simulink model "furuta_block_model_fixed_ppo_swingup"  (R2026b)
settings: Solver=ode14x  StopTime=25  FixedStep=driveElectrical.sampleTime
InitFcn:
  | validate_furuta_fixed_test(bdroot);
model workspace (MAT data in the model file):
  calibration = [73.65 -1 4058.5 1]
  controlPeriod = 0.01
  drive = [-1 1.5 1.5 inf]
  driveElectrical : object (value not decoded)
  failureReplayEnabled = 0
  failureReplaySlowdown = 10
  failureReplaySource = 'C:\Capstone1\matlab_furuta\results\ppo_rmd_candidate_tpa79dc374_f9fe_4d66_a12a_2e210f4a8415\ppo_start_-20_+20_armrate_20_current_1.5_time_10_armlimit_Inf.mat'
  failureReplayStartDeg = 20
  failureReplayState = [0 0.1 0.2 0.3 0.4 0.5 0.6 0.7 0.8 0.9 1 1.1 ... (205 elements, 41x5)]
  furutaPPOAgent : rl.agent.rlPPOAgent (value not decoded)
  furutaSACAgent : rl.agent.rlSACAgent (value not decoded)
  furutaToolboxMpc : object (value not decoded)
  initialState = [0; 3.14159265359; 0; 0]
  integrationStep = 0.002
  limits = [inf 3.3 15 20]
  lqrGain = [-1.90684760658 -25.0276005412 -1.03983138576 -2.50199272238]
  maxTorque = 3.15
  milVelocityLimits = [15 25]
  pidGains = [25.0276005412 5.00398544475 1.90684760658 2.07966277151 0.001]
  plantCoefficients = [0.05 0.00016078 0.00016134 0.00013805 0.016934 0.0001 1e-05 0.63]
  rlRewardLevel = 2
  rmd : object (value not decoded)
  rmdCommandDelaySamples = 1
  scenarioStimulus = [0  0  0  0; 20  0  0  0]
  swingLqrThresholds = [0.226892802759 0.2 0.523598775598]
  usePolicyCallback = 0
  useRmd = 1
  velocityFilterTau = 0.03
values from neighbouring files (symbols this model uses):
  C = [B A*B A^2*B A^3*B]    [build_furuta_rmd.m]
  N = 20    [build_furuta_rl.m]    (also in design_classical.m)
  s = load(matFile,'ds')    [analyze_pi_current_run.m]    (also in analyze_pi_speed_run.m; build_furuta_rl.m = sin(x(2));"; build_furuta_simulink.m = s(1); design_classical.m = furuta_scenarios)
  source = [step '/1']    [add_furuta_plant_blocks.m]    (also in build_furuta_pi.m = get_param(line,'SrcPortHandle'); build_furuta_pi_hardware.m = 'Drive interlocks/3'; compare_furuta_actuators.m = get_param([harness '/Requested torque'],'PortHandles'))
  Z = expm([A B; zeros(1,5)]*p.Ts)    [furuta_linearize.m]
symbols that are objects in the model workspace (value not decoded): driveElectrical, rmd
undefined symbols (not defined in the file or in its folder): lmpcF, lmpcH, poleGain, sgn, X, Y
libraries: sm_lib x36, raspberrypiCommlib x9, nesl_utility x8, fl_lib x7, rllib x2, mpclib x1, slpidlib x1, ee_lib x1
(part 4 of 4)

== system furuta_block_model_fixed_ppo_swingup/01 MIL - Controller and Plant/05 Furuta plant/RK4 Furuta plant/Substep 4/k3 ==
  x : Inport
  tau : Inport  Port=2
  Arm acceleration : Fcn  Expr=(u(3)*u(4)-u(2)*u(5))/(u(1)*u(3)-(u(2)*u(2)))
  Arm rate : Fcn  Expr=u(3)
  D11 : Fcn  Expr=u(6)+u(7)*(sin(u(2))*sin(u(2)))
  D12 : Fcn  Expr=u(9)*cos(u(2))
  D22 : Fcn  Expr=u(8)
  Mass matrix and RHS : Mux  Inputs=5
  Pend acceleration : Fcn  Expr=(u(1)*u(5)-u(2)*u(4))/(u(1)*u(3)-(u(2)*u(2)))
  Pend rate : Fcn  Expr=u(4)
  Physical parameters : Constant  Value=plantCoefficients
  State derivative : Mux
  State torque parameters : Mux  Inputs=3
  Torque RHS arm : Fcn  Expr=u(5)-2*u(7)*sin(u(2))*cos(u(2))*u(3)*u(4)+u(9)*sin(u(2))*(u(4)*u(4))-u(11)*u(3)-u(13)*sgn(u(3))
  Torque RHS pend : Fcn  Expr=u(7)*sin(u(2))*cos(u(2))*(u(3)*u(3))-u(12)*u(4)+u(10)*sin(u(2))
  xdot : Outport
  wires:
  x/1 -> State torque parameters/1
  tau/1 -> State torque parameters/2
  Physical parameters/1 -> State torque parameters/3
  State torque parameters/1 -> Arm rate/1, Pend rate/1, Torque RHS pend/1, Torque RHS arm/1, D22/1, D11/1, D12/1
  D11/1 -> Mass matrix and RHS/1
  D12/1 -> Mass matrix and RHS/2
  D22/1 -> Mass matrix and RHS/3
  Torque RHS arm/1 -> Mass matrix and RHS/4
  Torque RHS pend/1 -> Mass matrix and RHS/5
  Arm rate/1 -> State derivative/1
  Pend rate/1 -> State derivative/2
  Mass matrix and RHS/1 -> Arm acceleration/1, Pend acceleration/1
  Arm acceleration/1 -> State derivative/3
  Pend acceleration/1 -> State derivative/4
  State derivative/1 -> xdot/1

== system furuta_block_model_fixed_ppo_swingup/01 MIL - Controller and Plant/05 Furuta plant/RK4 Furuta plant/Substep 4/k4 ==
  x : Inport
  tau : Inport  Port=2
  Arm acceleration : Fcn  Expr=(u(3)*u(4)-u(2)*u(5))/(u(1)*u(3)-(u(2)*u(2)))
  Arm rate : Fcn  Expr=u(3)
  D11 : Fcn  Expr=u(6)+u(7)*(sin(u(2))*sin(u(2)))
  D12 : Fcn  Expr=u(9)*cos(u(2))
  D22 : Fcn  Expr=u(8)
  Mass matrix and RHS : Mux  Inputs=5
  Pend acceleration : Fcn  Expr=(u(1)*u(5)-u(2)*u(4))/(u(1)*u(3)-(u(2)*u(2)))
  Pend rate : Fcn  Expr=u(4)
  Physical parameters : Constant  Value=plantCoefficients
  State derivative : Mux
  State torque parameters : Mux  Inputs=3
  Torque RHS arm : Fcn  Expr=u(5)-2*u(7)*sin(u(2))*cos(u(2))*u(3)*u(4)+u(9)*sin(u(2))*(u(4)*u(4))-u(11)*u(3)-u(13)*sgn(u(3))
  Torque RHS pend : Fcn  Expr=u(7)*sin(u(2))*cos(u(2))*(u(3)*u(3))-u(12)*u(4)+u(10)*sin(u(2))
  xdot : Outport
  wires:
  x/1 -> State torque parameters/1
  tau/1 -> State torque parameters/2
  Physical parameters/1 -> State torque parameters/3
  State torque parameters/1 -> Arm rate/1, Pend rate/1, Torque RHS pend/1, Torque RHS arm/1, D22/1, D11/1, D12/1
  D11/1 -> Mass matrix and RHS/1
  D12/1 -> Mass matrix and RHS/2
  D22/1 -> Mass matrix and RHS/3
  Torque RHS arm/1 -> Mass matrix and RHS/4
  Torque RHS pend/1 -> Mass matrix and RHS/5
  Arm rate/1 -> State derivative/1
  Pend rate/1 -> State derivative/2
  Mass matrix and RHS/1 -> Arm acceleration/1, Pend acceleration/1
  Arm acceleration/1 -> State derivative/3
  Pend acceleration/1 -> State derivative/4
  State derivative/1 -> xdot/1

== system furuta_block_model_fixed_ppo_swingup/01 MIL - Controller and Plant/05 Furuta plant/RK4 Furuta plant/Substep 5/k1 ==
  x : Inport
  tau : Inport  Port=2
  Arm acceleration : Fcn  Expr=(u(3)*u(4)-u(2)*u(5))/(u(1)*u(3)-(u(2)*u(2)))
  Arm rate : Fcn  Expr=u(3)
  D11 : Fcn  Expr=u(6)+u(7)*(sin(u(2))*sin(u(2)))
  D12 : Fcn  Expr=u(9)*cos(u(2))
  D22 : Fcn  Expr=u(8)
  Mass matrix and RHS : Mux  Inputs=5
  Pend acceleration : Fcn  Expr=(u(1)*u(5)-u(2)*u(4))/(u(1)*u(3)-(u(2)*u(2)))
  Pend rate : Fcn  Expr=u(4)
  Physical parameters : Constant  Value=plantCoefficients
  State derivative : Mux
  State torque parameters : Mux  Inputs=3
  Torque RHS arm : Fcn  Expr=u(5)-2*u(7)*sin(u(2))*cos(u(2))*u(3)*u(4)+u(9)*sin(u(2))*(u(4)*u(4))-u(11)*u(3)-u(13)*sgn(u(3))
  Torque RHS pend : Fcn  Expr=u(7)*sin(u(2))*cos(u(2))*(u(3)*u(3))-u(12)*u(4)+u(10)*sin(u(2))
  xdot : Outport
  wires:
  State derivative/1 -> xdot/1
  Pend acceleration/1 -> State derivative/4
  Arm acceleration/1 -> State derivative/3
  Mass matrix and RHS/1 -> Pend acceleration/1, Arm acceleration/1
  Pend rate/1 -> State derivative/2
  Arm rate/1 -> State derivative/1
  Torque RHS pend/1 -> Mass matrix and RHS/5
  Torque RHS arm/1 -> Mass matrix and RHS/4
  D22/1 -> Mass matrix and RHS/3
  D12/1 -> Mass matrix and RHS/2
  D11/1 -> Mass matrix and RHS/1
  State torque parameters/1 -> Pend rate/1, Arm rate/1, Torque RHS pend/1, Torque RHS arm/1, D22/1, D12/1, D11/1
  Physical parameters/1 -> State torque parameters/3
  tau/1 -> State torque parameters/2
  x/1 -> State torque parameters/1

== system furuta_block_model_fixed_ppo_swingup/01 MIL - Controller and Plant/05 Furuta plant/RK4 Furuta plant/Substep 5/k2 ==
  x : Inport
  tau : Inport  Port=2
  Arm acceleration : Fcn  Expr=(u(3)*u(4)-u(2)*u(5))/(u(1)*u(3)-(u(2)*u(2)))
  Arm rate : Fcn  Expr=u(3)
  D11 : Fcn  Expr=u(6)+u(7)*(sin(u(2))*sin(u(2)))
  D12 : Fcn  Expr=u(9)*cos(u(2))
  D22 : Fcn  Expr=u(8)
  Mass matrix and RHS : Mux  Inputs=5
  Pend acceleration : Fcn  Expr=(u(1)*u(5)-u(2)*u(4))/(u(1)*u(3)-(u(2)*u(2)))
  Pend rate : Fcn  Expr=u(4)
  Physical parameters : Constant  Value=plantCoefficients
  State derivative : Mux
  State torque parameters : Mux  Inputs=3
  Torque RHS arm : Fcn  Expr=u(5)-2*u(7)*sin(u(2))*cos(u(2))*u(3)*u(4)+u(9)*sin(u(2))*(u(4)*u(4))-u(11)*u(3)-u(13)*sgn(u(3))
  Torque RHS pend : Fcn  Expr=u(7)*sin(u(2))*cos(u(2))*(u(3)*u(3))-u(12)*u(4)+u(10)*sin(u(2))
  xdot : Outport
  wires:
  x/1 -> State torque parameters/1
  tau/1 -> State torque parameters/2
  Physical parameters/1 -> State torque parameters/3
  State torque parameters/1 -> Arm rate/1, Pend rate/1, Torque RHS pend/1, Torque RHS arm/1, D22/1, D11/1, D12/1
  D11/1 -> Mass matrix and RHS/1
  D12/1 -> Mass matrix and RHS/2
  D22/1 -> Mass matrix and RHS/3
  Torque RHS arm/1 -> Mass matrix and RHS/4
  Torque RHS pend/1 -> Mass matrix and RHS/5
  Arm rate/1 -> State derivative/1
  Pend rate/1 -> State derivative/2
  Mass matrix and RHS/1 -> Arm acceleration/1, Pend acceleration/1
  Arm acceleration/1 -> State derivative/3
  Pend acceleration/1 -> State derivative/4
  State derivative/1 -> xdot/1

== system furuta_block_model_fixed_ppo_swingup/01 MIL - Controller and Plant/05 Furuta plant/RK4 Furuta plant/Substep 5/k3 ==
  x : Inport
  tau : Inport  Port=2
  Arm acceleration : Fcn  Expr=(u(3)*u(4)-u(2)*u(5))/(u(1)*u(3)-(u(2)*u(2)))
  Arm rate : Fcn  Expr=u(3)
  D11 : Fcn  Expr=u(6)+u(7)*(sin(u(2))*sin(u(2)))
  D12 : Fcn  Expr=u(9)*cos(u(2))
  D22 : Fcn  Expr=u(8)
  Mass matrix and RHS : Mux  Inputs=5
  Pend acceleration : Fcn  Expr=(u(1)*u(5)-u(2)*u(4))/(u(1)*u(3)-(u(2)*u(2)))
  Pend rate : Fcn  Expr=u(4)
  Physical parameters : Constant  Value=plantCoefficients
  State derivative : Mux
  State torque parameters : Mux  Inputs=3
  Torque RHS arm : Fcn  Expr=u(5)-2*u(7)*sin(u(2))*cos(u(2))*u(3)*u(4)+u(9)*sin(u(2))*(u(4)*u(4))-u(11)*u(3)-u(13)*sgn(u(3))
  Torque RHS pend : Fcn  Expr=u(7)*sin(u(2))*cos(u(2))*(u(3)*u(3))-u(12)*u(4)+u(10)*sin(u(2))
  xdot : Outport
  wires:
  x/1 -> State torque parameters/1
  tau/1 -> State torque parameters/2
  Physical parameters/1 -> State torque parameters/3
  State torque parameters/1 -> Arm rate/1, Pend rate/1, Torque RHS pend/1, Torque RHS arm/1, D22/1, D11/1, D12/1
  D11/1 -> Mass matrix and RHS/1
  D12/1 -> Mass matrix and RHS/2
  D22/1 -> Mass matrix and RHS/3
  Torque RHS arm/1 -> Mass matrix and RHS/4
  Torque RHS pend/1 -> Mass matrix and RHS/5
  Arm rate/1 -> State derivative/1
  Pend rate/1 -> State derivative/2
  Mass matrix and RHS/1 -> Arm acceleration/1, Pend acceleration/1
  Arm acceleration/1 -> State derivative/3
  Pend acceleration/1 -> State derivative/4
  State derivative/1 -> xdot/1

== system furuta_block_model_fixed_ppo_swingup/01 MIL - Controller and Plant/05 Furuta plant/RK4 Furuta plant/Substep 5/k4 ==
  x : Inport
  tau : Inport  Port=2
  Arm acceleration : Fcn  Expr=(u(3)*u(4)-u(2)*u(5))/(u(1)*u(3)-(u(2)*u(2)))
  Arm rate : Fcn  Expr=u(3)
  D11 : Fcn  Expr=u(6)+u(7)*(sin(u(2))*sin(u(2)))
  D12 : Fcn  Expr=u(9)*cos(u(2))
  D22 : Fcn  Expr=u(8)
  Mass matrix and RHS : Mux  Inputs=5
  Pend acceleration : Fcn  Expr=(u(1)*u(5)-u(2)*u(4))/(u(1)*u(3)-(u(2)*u(2)))
  Pend rate : Fcn  Expr=u(4)
  Physical parameters : Constant  Value=plantCoefficients
  State derivative : Mux
  State torque parameters : Mux  Inputs=3
  Torque RHS arm : Fcn  Expr=u(5)-2*u(7)*sin(u(2))*cos(u(2))*u(3)*u(4)+u(9)*sin(u(2))*(u(4)*u(4))-u(11)*u(3)-u(13)*sgn(u(3))
  Torque RHS pend : Fcn  Expr=u(7)*sin(u(2))*cos(u(2))*(u(3)*u(3))-u(12)*u(4)+u(10)*sin(u(2))
  xdot : Outport
  wires:
  x/1 -> State torque parameters/1
  tau/1 -> State torque parameters/2
  Physical parameters/1 -> State torque parameters/3
  State torque parameters/1 -> Arm rate/1, Pend rate/1, Torque RHS pend/1, Torque RHS arm/1, D22/1, D11/1, D12/1
  D11/1 -> Mass matrix and RHS/1
  D12/1 -> Mass matrix and RHS/2
  D22/1 -> Mass matrix and RHS/3
  Torque RHS arm/1 -> Mass matrix and RHS/4
  Torque RHS pend/1 -> Mass matrix and RHS/5
  Arm rate/1 -> State derivative/1
  Pend rate/1 -> State derivative/2
  Mass matrix and RHS/1 -> Arm acceleration/1, Pend acceleration/1
  Arm acceleration/1 -> State derivative/3
  Pend acceleration/1 -> State derivative/4
  State derivative/1 -> xdot/1

== matlab function furuta_block_model_fixed_ppo_swingup/03 Pi - Motor Control and Telemetry/Sensor decoder ==
  data: frame input; obs output; status input; err input; remote input; magnet input; mstat input; angle input; astat input; cal input; act input; valid output; act output; ack output
function [obs,valid,act, ack] = decode(frame,status,err,remote,magnet,mstat,angle,astat,cal,act)
[obs,valid,ack] = furuta_pi_sample(frame,status,err,remote,magnet,mstat,angle,astat,cal,act);
end

== matlab function furuta_block_model_fixed_ppo_swingup/03 Pi - Motor Control and Telemetry/Telemetry ==
  data: requested input; obs input; valid input; act input; ack input; a input; t input; packet input; row output
function row = logrow(requested,obs,valid,act,ack,a,t, packet)
row = [t; double(act); double(valid); obs; a; double(packet(1)); double(ack); requested];
end

== matlab function furuta_block_model_fixed_ppo_swingup/02 Pi - Sensor and RMD Diagnostics/Bench diagnostics ==
  data: frame input; electrical output; rx input; err input; remote input; mag input; ms input; angle input; as input; cal input; query input; expected input; angles output; health output
function [electrical,angles,health] = diagnostics(frame,rx,err,remote,mag,ms,angle,as,cal,query,expected)
[electrical,angles,health] = furuta_pi_verify_sample(frame,rx,err,remote,mag,ms,angle,as,cal,query,expected);
end

== matlab function furuta_block_model_fixed_ppo_swingup/02 Pi - Sensor and RMD Diagnostics/Read-only CAN schedule ==
  data: query output; t input; packet output; expected output
function [query,packet,expected] = schedule(t)
tick = round(t/.005);
codes = uint8([146 154 156]);
expected = codes(mod(floor(tick/2),3)+1);
query = mod(tick,2)==0;
packet = [expected zeros(1,7,'uint8')];
end

== matlab function furuta_block_model_fixed_ppo_swingup/04 PC - Functional Self-Test/Compare with expected ==
  data: n input; pass output; packet input; send input; actual input; valid input; row output
function [pass,row] = compare(n,packet,send,actual,valid)
expectedOpcode = uint8([0 161 161 128 128 128]);
expectedLow = uint8([0 10 246 0 0 0]);
expectedHigh = uint8([0 0 255 0 0 0]);
expectedAction = [0 .1 -.1 0 0 0];
expectedValid = [false true true false false true];
i = n+1;
expected = [expectedOpcode(i) 0 0 0 expectedLow(i) expectedHigh(i) 0 0];
pass = all(packet==expected) && send==(n~=0) && actual==expectedAction(i) && valid==expectedValid(i);
row = [n;double(pass);double(packet(1));actual;double(valid)];
end

== matlab function furuta_block_model_fixed_ppo_swingup/04 PC - Functional Self-Test/Furuta blocks under test ==
  data: arm input; packet output; rx input; a input; enable input; send output; actual output; valid output
function [packet,send,actual,valid] = test(arm,rx,a,enable)
[o,valid] = furuta_pi_decode(arm,rx,uint8(32),uint8([15 219]),[-209.05 -1 4058.5 1],.01);
[packet,send,actual] = furuta_pi_frame(a,o,valid,enable,1,1,.1,ones(1,4),0,1);
end

== matlab function furuta_block_model_fixed_ppo_swingup/04 PC - Functional Self-Test/Test sequence ==
  data: t input; n output; arm output; rx output; action output; enable output
function [n,arm,rx,action,enable] = cases(t)
n = min(5,round(t/.01));
arm = uint8([146 0 0 0 87 174 255 255]);
rx = n~=3;
action = 1-2*double(n==2);
enable = n~=0;
end

== matlab function furuta_block_model_fixed_ppo_swingup/03 Pi - Motor Control and Telemetry/PPO shadow telemetry ==
  data: requested input; action output; obs input; valid input; enabled input
function action = shadow(requested,obs,valid,enabled)
action = requested;
if enabled
    action = NaN;
    if valid && all(isfinite(obs))
        action = infer(obs);
    end
end
end
function a = infer(obs)
h = tanh([0.21985654532909393 0.0095907049253582954 0.25029578804969788 0.059855211526155472 0.15152357518672943;-0.19411937892436981 0.036094587296247482 -0.045075841248035431 0.306905597448349 -0.22275532782077789;0.026761472225189209 -0.061149749904870987 0.15520088374614716 -0.024567000567913055 0.019287874922156334;0.21795064210891724 0.098515421152114868 -0.17018890380859375 0.029285585507750511 -0.27904951572418213;-0.27294778823852539 0.030370831489562988 -0.1757798045873642 0.17474332451820374 -0.085558339953422546;0.14998310804367065 0.040673054754734039 0.056430410593748093 0.30176636576652527 0.095863170921802521;0.061508547514677048 0.035619847476482391 0.065281808376312256 -0.15538105368614197 -0.097707860171794891;0.30632543563842773 -0.012846404686570168 0.18552382290363312 -0.21049897372722626 -0.17877112329006195;0.089963190257549286 0.084782369434833527 0.25272056460380554 0.35577654838562012 0.32066875696182251;-0.31001079082489014 0.15277655422687531 0.24734412133693695 0.26968944072723389 0.32205238938331604;0.13535942137241364 0.0012935638660565019 0.027015933766961098 -0.18284960091114044 -0.078767813742160797;-0.0004048009286634624 -0.035848449915647507 -0.14923247694969177 0.22261823713779449 0.089110620319843292;0.05899394303560257 -0.040005188435316086 -0.037826143205165863 0.086127288639545441 -0.15595641732215881;0.30924123525619507 0.032104413956403732 -0.13415318727493286 -0.22335295379161835 -0.36496090888977051;0.31227928400039673 -0.17364141345024109 -0.02787318266928196 -0.075402267277240753 -0.32210990786552429;-0.051128581166267395 0.13989441096782684 -0.056596137583255768 -0.07464328408241272 0.13918361067771912;-0.13320431113243103 0.036680798977613449 0.05425991490483284 0.32326355576515198 0.29038485884666443;-0.011552967131137848 0.054514821618795395 0.25109755992889404 -0.15508747100830078 -0.031780753284692764;-0.053429316729307175 0.0070675746537744999 0.093582980334758759 -0.2984592616558075 0.027203243225812912;0.15923863649368286 0.059559609740972519 -0.086173936724662781 -0.012859993614256382 0.29073435068130493;-0.058516938239336014 0.15989454090595245 -0.0040564159862697124 -0.13487106561660767 -0.11496218293905258;-0.17286650836467743 -0.0098589388653635979 -0.013808916322886944 0.046467162668704987 0.023124983534216881;0.033895567059516907 0.017516924068331718 -0.1770862489938736 -0.20185215771198273 -0.067111864686012268;-0.24703015387058258 0.028943369165062904 -0.024457771331071854 0.15350465476512909 -0.067847996950149536;0.2409043163061142 -0.009560353122651577 -0.10825634002685547 0.057186368852853775 0.078938789665699005;0.029955318197607994 -0.025293624028563499 -0.33040258288383484 0.096989616751670837 0.020557217299938202;0.23130552470684052 0.026648884639143944 -0.032627295702695847 -0.085689567029476166 -0.10357806086540222;-0.23711241781711578 0.042608395218849182 -0.030292246490716934 -0.17892241477966309 -0.036687444895505905;-0.12672953307628632 0.10810898989439011 0.13519139587879181 0.35656663775444031 0.012146779336035252;0.021120971068739891 -0.22286206483840942 0.15575708448886871 0.16309067606925964 0.15226514637470245;-0.27690857648849487 0.0059896400198340416 0.22356896102428436 0.066083826124668121 0.31826218962669373;0.30257150530815125 -0.00093157921219244599 0.087923601269721985 0.21082617342472076 0.31943482160568237]*obs+[-0.030704321339726448;0.036847405135631561;-0.021215939894318581;-0.008288772776722908;0.062692493200302124;-0.012231994420289993;-0.035373415797948837;-0.055833209306001663;-0.0063572614453732967;0.020074689760804176;-0.039045251905918121;0.0049597811885178089;0.00021228115656413138;-0.019910916686058044;-0.017786165699362755;-0.00095275416970252991;0.014119599014520645;-0.005820159800350666;0.0036877458915114403;-0.05056096613407135;0.0083994520828127861;0.061484746634960175;-0.012749716639518738;0.068205393850803375;-0.05071287602186203;-0.0017137343529611826;-0.037252165377140045;0.021494664251804352;0.020272744819521904;-0.00012999310274608433;0.012779717333614826;-0.030294071882963181]);
a = tanh([-0.00097632699180394411 7.2949185371398926 0.56279486417770386 0.30360612273216248 0.69415199756622314]*obs+(-0.00098355580121278763)+[-0.0016546585829928517 0.0040160287171602249 -0.0026487153954803944 -0.00093255285173654556 0.0024696481414139271 0.001415426260791719 0.00028291609487496316 -0.00086479476885870099 0.0028804875910282135 0.00056480569764971733 -0.00087148119928315282 0.0014196488773450255 -0.00067392515484243631 -5.1617509598145261e-05 -0.0018752050818875432 0.0010691009229049087 0.0017207276541739702 -0.00026108429301530123 -0.0030731367878615856 -0.0014377455227077007 0.0021921882871538401 2.883478555304464e-05 -0.001404054113663733 0.0019714981317520142 -0.00033255116431973875 0.0010078819468617439 7.792503311065957e-06 0.00095984805375337601 0.0044766711071133614 0.0033149169757962227 0.0012992238625884056 -0.0013119500363245606]*h+(-0.00098355580121278763));
end

== matlab function furuta_block_model_fixed_ppo_swingup/01 MIL - Controller and Plant/03 Controllers/PID/PID with anti windup ==
  data: x input; u output; g input; dt input; mode input
function u = pid(x,g,dt,mode)
% 적분은 PID 모드에서만 갱신하고 입력 포화 방향에서는 누적하지 않는다.
persistent integral
if isempty(integral) || mode ~= 0
    integral = 0;
end
e = atan2(sin(x(2)),cos(x(2)));
base = g(1)*e+g(2)*x(4)+g(3)*x(1)+g(4)*x(3);
candidate = base+g(5)*(integral+dt*e);
if mode == 0 && (abs(candidate)<=1 || sign(candidate)~=sign(e))
    integral = integral+dt*e;
end
u = base+g(5)*integral;
end

== matlab function furuta_block_model_fixed_ppo_swingup/01 MIL - Controller and Plant/03 Controllers/LQR/Swing-up to LQR ==
  data: x input; u output; balance input; mode input; thresholds input; p input; balancing output
function [u,balancing]=control(x,balance,mode,thresholds,p)
[u,balancing]=furuta_swing_lqr_step(x,balance,mode==1,thresholds,p,0);
end

== matlab function furuta_block_model_fixed_ppo_swingup/01 MIL - Controller and Plant/03 Controllers/LQR/Capture arm reference ==
  data: x input; relative output; mode input; thresholds input; gatedMode output; home output
function [relative,gatedMode,home]=reference(x,mode,thresholds)
[relative,balancing,home]=furuta_balance_reference(x,mode==1,thresholds);
gatedMode=-1; if balancing, gatedMode=mode; end
end

== matlab function furuta_block_model_fixed_ppo_swingup/01 MIL - Controller and Plant/03 Controllers/PID/Swing-up to PID ==
  data: x input; u output; balance input; mode input; thresholds input; p input; balancing output
function [u,balancing]=control(x,balance,mode,thresholds,p)
[u,balancing]=furuta_swing_lqr_step(x,balance,mode==0,thresholds,p,0);
end

== matlab function furuta_block_model_fixed_ppo_swingup/01 MIL - Controller and Plant/03 Controllers/PID/Capture arm reference ==
  data: x input; relative output; mode input; thresholds input; gatedMode output; home output
function [relative,gatedMode,home]=reference(x,mode,thresholds)
[relative,balancing,home]=furuta_balance_reference(x,mode==0,thresholds);
gatedMode=-1; if balancing, gatedMode=mode; end
end

== matlab function furuta_block_model_fixed_ppo_swingup/01 MIL - Controller and Plant/06 Monitoring/MIL velocity guard ==
  data: x input; stop output; limits input
function stop=guard(x,limits)
stop=any(~isfinite(x)) || abs(x(3))>=limits(1) || abs(x(4))>=limits(2);
end

== matlab function furuta_block_model_fixed_ppo_swingup/01 MIL - Controller and Plant/03 Controllers/SAC/RL observation reward termination ==
  data: x input; obs output; lastAction input; level input; mode input; reward output; done output
function [obs,reward,done] = observe(x,lastAction,level,mode)
% 상태는 현재 샘플, 보상에 쓰는 행동은 이전 샘플이다.
stateVector = x(:);
active = mode == 4;
obs = zeros(5,1);
reward = 0;
done = false;
if ~active
    return
end
persistent startedUpright
if isempty(startedUpright)
    startedUpright = abs(atan2(sin(stateVector(2)),cos(stateVector(2))))<pi/9;
end
angle = abs(atan2(sin(stateVector(2)),cos(stateVector(2))));
if any(~isfinite(stateVector)) || abs(stateVector(1))>2*pi || max(abs(stateVector(3:4)))>30 || (startedUpright && angle>pi/4)
    done = true;
    reward = -50;
    return
end
c = cos(x(2)); s = sin(x(2));
obs = [c;s;x(1);x(3);x(4)];
reward = c-0.01*lastAction^2;
if level == 2
    reward = reward-.001*x(4)^2-.00002*x(3)^2+double(abs(atan2(s,c))<.35);
end
done = mode == 4 && abs(x(1))>2*pi;
if done
    reward = -50;
end
end

== matlab function furuta_block_model_fixed_ppo_swingup/03 Pi - Motor Control and Telemetry/CAN slots ==
  data: t input; query output; act output
function [query,act] = slots(t)
act = mod(round(t/.005),2)==1;
query = ~act;
end

== matlab function furuta_block_model_fixed_ppo_swingup/01 MIL - Controller and Plant/03 Controllers/LMPC (sim)/LMPC bounded QP ==
  data: x input; u output; mode input; H input; F input
function u = move(x,mode,H,F)
% 이전 해를 한 단계 이동해 재사용하고 모든 좌표를 [-1,1]로 제한한다.
persistent previous
if isempty(previous)
    previous = zeros(20,1);
end
u = 0;
if mode ~= 6
    previous(:) = 0;
    return
end
z = x(:);
z(2) = atan2(sin(z(2)),cos(z(2)));
f = F*z;
U = [previous(2:end); previous(end)];
gradient = H*U+f;
for it = 1:100
    change = 0;
    for j = 1:20
        next = min(1,max(-1,U(j)-gradient(j)/H(j,j)));
        step = next-U(j);
        U(j) = next;
        gradient = gradient+H(:,j)*step;
        change = max(change,abs(step));
    end
    if change<1e-7
        break
    end
end
previous = U;
u = U(1);
end

== matlab function furuta_block_model_fixed_ppo_swingup/01 MIL - Controller and Plant/04 Actuator/RMD X6 P20 60 E/01 RMD Driver/Current PI and duty ==
  data: reference input; duty output; current input; emf input; p input; v output
function [duty,v] = regulate(reference,current,emf,p)
% 3상 등가 q축 전압 제한으로 정규화한 평균 브리지 지령.
persistent integral
if isempty(integral)
    integral = 0;
end
err = reference-current;
raw = emf+p(1)*err+integral;
vmax = p(4)/sqrt(3);
v = max(-vmax,min(vmax,raw));
if abs(raw)<=vmax || sign(raw)~=sign(err)
    integral = integral+p(2)*p(3)*err;
end
duty = .5+.5*v/p(4);
end

== matlab function furuta_block_model_fixed_ppo_swingup/03 Pi - Motor Control and Telemetry/Drive interlocks ==
  data: obs output; valid output; act output; ack output; applied output; t output; packet output; send output; a input; obs input; valid input; act input; ack input; d input; lim input; t input
function [obs, valid, act, ack,applied, t,packet, send] = command(a,obs,valid,act,ack,d,lim,t)
persistent needsAck count
if isempty(needsAck), needsAck = false; count = 0; end
packet = zeros(1,8,'uint8'); send = false; applied = 0;
if ~act || d(4)==0, return, end
if valid, count = count+1; end
engaged = count>0 || t>.2;
[packet,send,applied] = furuta_pi_frame(a,obs,valid && (~needsAck || ack),engaged,d(1),d(2),d(3),lim,t,d(4));
needsAck = packet(1)==161;

end

== matlab function furuta_block_model_fixed_ppo_swingup/01 MIL - Controller and Plant/03 Controllers/PPO/RL observation reward termination ==
  data: x input; obs output; lastAction input; level input; mode input; reward output; done output
function [obs,reward,done] = observe(x,lastAction,level,mode)
% 상태는 현재 샘플, 보상에 쓰는 행동은 이전 샘플이다.
stateVector = mode(:);
active = x == 3;
obs = zeros(5,1);
reward = 0;
done = false;
if ~active
    return
end
persistent startedUpright
if isempty(startedUpright)
    startedUpright = abs(atan2(sin(stateVector(2)),cos(stateVector(2))))<pi/9;
end
angle = abs(atan2(sin(stateVector(2)),cos(stateVector(2))));
if any(~isfinite(stateVector)) || max(abs(stateVector(3:4)))>30 || (startedUpright && angle>pi/4)
    done = true;
    reward = -50;
    return
end
c = cos(mode(2)); s = sin(mode(2));
obs = [c;s;atan2(sin(mode(1)),cos(mode(1)));mode(3);mode(4)];
reward = c-0.01*lastAction^2;
if level == 2
    reward = reward-.001*mode(4)^2-.00002*mode(3)^2+double(abs(atan2(s,c))<.35);
end
done = false;
if done
    reward = -50;
end
end
